simulink model "hdlcoder_fft40"  (R2026a)
settings: Solver=FixedStepDiscrete  StopTime=stoptime
PostLoadFcn:
  | load('fft40_vars.mat')
values from neighbouring files (symbols this model uses):
  N = 40    [fft40_vars.mat]
undefined symbols (not defined in the file or in its folder): TWIDDLE
libraries: dsphdlxfrm x5, dspsrcs4 x2
settings Model: DataTypeOverride=Off  Creator=The MathWorks, Inc.  LastModifiedBy=The MathWorks, Inc.
settings OptimizationCC: ConditionallyExecuteInputs=off
settings DebuggingCC: SignalRangeChecking=warning  AlgebraicLoopMsg=error  SingleTaskRateTransMsg=error  PregeneratedLibrarySubsystemCodeDiagnostic=none
settings HardwareCC: ProdHWDeviceType=ASIC/FPGA->ASIC/FPGA  TargetBitPerLong=64.0  TargetBitPerPointer=64.0  TargetBitPerSizeT=64.0  TargetBitPerPtrDiffT=64.0  TargetLongLongMode=on  TargetIntDivRoundTo=Zero  TargetEndianess=LittleEndian  TargetWordSize=64.0  TargetHWDeviceType=Custom Processor->MATLAB Host Computer  ProdEqTarget=off

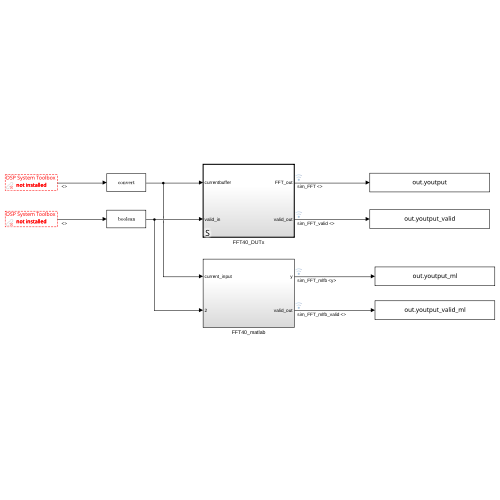
[thumbnail: Simulink's stored preview of the top-level diagram]
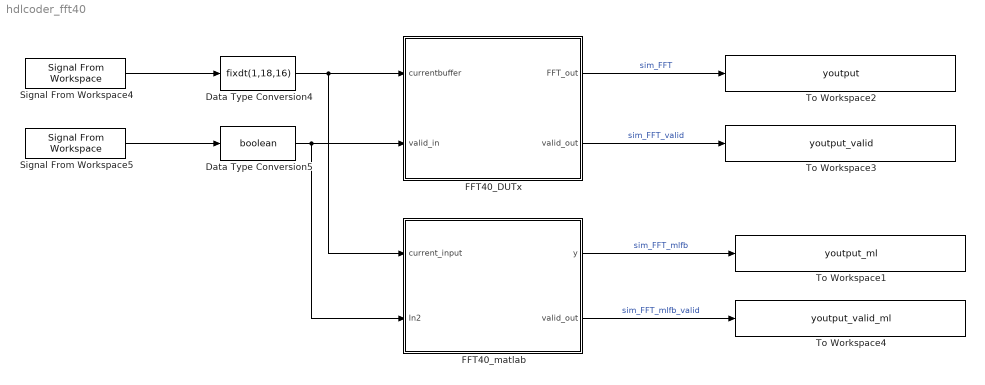
== system hdlcoder_fft40 ==
  Data Type Conversion4 : DataTypeConversion  OutDataTypeStr=fixdt(1,18,16)  SaturateOnIntegerOverflow=off  RndMeth=Floor
  Data Type Conversion5 : DataTypeConversion  OutDataTypeStr=boolean  SaturateOnIntegerOverflow=off  RndMeth=Floor
  FFT40_DUTx : Subsystem
  FFT40_matlab : Subsystem
  Signal From Workspace4 : dspsrcs4/Signal From Workspace  X=xinput  Ts=1/N  nsamps=N  OutputAfterFinalValue=Setting to zero  ignoreOrWarnInputAndFrameLengths=off  OutputFrames=off
  Signal From Workspace5 : dspsrcs4/Signal From Workspace  X=xvalid  Ts=1  nsamps=1  OutputAfterFinalValue=Holding final value  ignoreOrWarnInputAndFrameLengths=off  OutputFrames=off
  To Workspace1 : ToWorkspace  VariableName=youtput_ml  SampleTime=-1
  To Workspace2 : ToWorkspace  VariableName=youtput  SampleTime=-1
  To Workspace3 : ToWorkspace  VariableName=youtput_valid  SampleTime=-1
  To Workspace4 : ToWorkspace  VariableName=youtput_valid_ml  SampleTime=-1
  wires:
  Data Type Conversion5/1 -> FFT40_matlab/2(In2), FFT40_DUTx/2(valid_in)
  Signal From Workspace5/1 -> Data Type Conversion5/1
  Data Type Conversion4/1 -> FFT40_matlab/1(current_input), FFT40_DUTx/1(currentbuffer)
  Signal From Workspace4/1 -> Data Type Conversion4/1
  FFT40_DUTx/2(valid_out) -> To Workspace3/1  "sim_FFT_valid"
  FFT40_DUTx/1(FFT_out) -> To Workspace2/1  "sim_FFT"
  FFT40_matlab/1(y) -> To Workspace1/1  "sim_FFT_mlfb"
  FFT40_matlab/2(valid_out) -> To Workspace4/1  "sim_FFT_mlfb_valid"

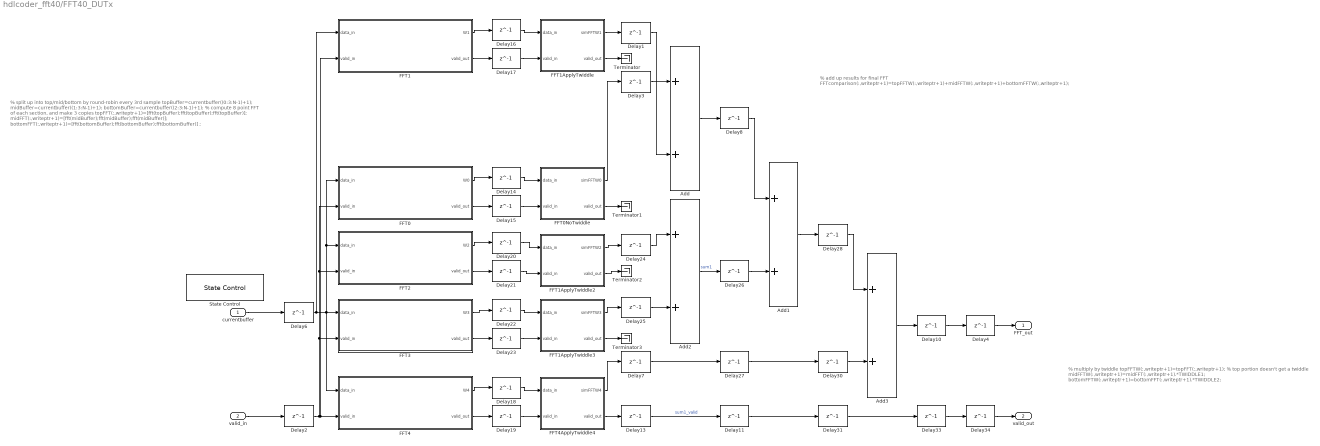
== system hdlcoder_fft40/FFT40_DUTx ==
  note: % split up into top/mid/bottom by round-robin every 3rd sample
      | topBuffer=currentbuffer((0:3:N-1)+1);
      | midBuffer=currentbuffer((1:3:N-1)+1);
      | bottomBuffer=currentbuffer((2:3:N-1)+1);
      |
      | % compute 8 point FFT of each section, and make 3 copies
      | topFFT(:,writeptr+1)=[fft(topBuffer);fft(topBuffer);fft(topBuffer)];
      | midFFT(:,writeptr+1)=[fft(midBuffer);fft(midBuffer);fft(midBuffer)];
      | bottomFFT(:,writeptr+1)=[fft(bottomBuffer);fft(bottomBuffer);fft(bottomBuffer)] ;
  note: % multiply by twiddle
      | topFFTW(:,writeptr+1)=topFFT(:,writeptr+1); % top portion doesn't get a twiddle
      | midFFTW(:,writeptr+1)=midFFT(:,writeptr+1).*TWIDDLE1;
      | bottomFFTW(:,writeptr+1)=bottomFFT(:,writeptr+1).*TWIDDLE2;
  note: % add up results for final FFT
      | FFTcomparison(:,writeptr+1)=topFFTW(:,writeptr+1)+midFFTW(:,writeptr+1)+bottomFFTW(:,writeptr+1);
  currentbuffer : Inport
  valid_in : Inport  Port=2
  Add{,1..3} (4 alike) : Sum
  Delay{1..4,6..8,10..11,13..28,30..31,33..34} (29 alike) : Delay  DelayLength=1  InitialCondition=0  UseCircularBuffer=on
  FFT0 : Subsystem
  FFT0NoTwiddle : Subsystem
  FFT1 : Subsystem
  FFT1ApplyTwiddle : Subsystem
  FFT1ApplyTwiddle2 : Subsystem
  FFT1ApplyTwiddle3 : Subsystem
  FFT2 : Subsystem
  FFT3 : Subsystem
  FFT4 : Subsystem
  FFT4ApplyTwiddle4 : Subsystem
  State Control : StateControl  StateControl=Synchronous
  Terminator{,1..3} (4 alike) : Terminator
  FFT_out : Outport
  valid_out : Outport  Port=2
  wires:
  Delay19/1 -> FFT4ApplyTwiddle4/2(valid_in)
  FFT4/1(W4) -> Delay18/1
  Delay20/1 -> FFT1ApplyTwiddle2/1(data_in)
  Add2/1 -> Delay26/1  "sum1"
  Delay1/1 -> Add/2
  Delay25/1 -> Add2/2
  Delay26/1 -> Add1/2
  Delay33/1 -> Delay34/1
  Add3/1 -> Delay10/1
  Delay24/1 -> Add2/1
  FFT3/2(valid_out) -> Delay23/1
  Delay2/1 -> FFT1/2(valid_in), FFT4/2(valid_in), FFT2/2(valid_in), FFT0/2(valid_in), FFT3/2(valid_in)
  FFT2/1(W2) -> Delay20/1
  Delay23/1 -> FFT1ApplyTwiddle3/2(valid_in)
  FFT1/2(valid_out) -> Delay17/1
  currentbuffer/1 -> Delay6/1
  FFT1ApplyTwiddle3/2(valid_out) -> Terminator3/1
  FFT1ApplyTwiddle2/2(valid_out) -> Terminator2/1
  Delay15/1 -> FFT0NoTwiddle/2(valid_in)
  FFT0NoTwiddle/2(valid_out) -> Terminator1/1
  FFT3/1(W3) -> Delay22/1
  FFT1ApplyTwiddle3/1(simFFTW3) -> Delay25/1
  FFT1ApplyTwiddle/2(valid_out) -> Terminator/1
  Delay4/1 -> FFT_out/1
  FFT1ApplyTwiddle2/1(simFFTW2) -> Delay24/1
  Delay16/1 -> FFT1ApplyTwiddle/1(data_in)
  FFT4ApplyTwiddle4/2(valid_out) -> Delay13/1
  FFT4/2(valid_out) -> Delay19/1
  Delay18/1 -> FFT4ApplyTwiddle4/1(data_in)
  Delay14/1 -> FFT0NoTwiddle/1(data_in)
  Delay10/1 -> Delay4/1
  FFT0/2(valid_out) -> Delay15/1
  valid_in/1 -> Delay2/1
  Delay8/1 -> Add1/1
  FFT4ApplyTwiddle4/1(simFFTW4) -> Delay7/1
  Delay3/1 -> Add/1
  FFT1/1(W1) -> Delay16/1
  Delay6/1 -> FFT0/1(data_in), FFT2/1(data_in), FFT3/1(data_in), FFT4/1(data_in), FFT1/1(data_in)
  FFT1ApplyTwiddle/1(simFFTW1) -> Delay1/1
  Delay17/1 -> FFT1ApplyTwiddle/2(valid_in)
  Delay21/1 -> FFT1ApplyTwiddle2/2(valid_in)
  Delay30/1 -> Add3/2
  Add1/1 -> Delay28/1
  FFT0/1(W0) -> Delay14/1
  Delay34/1 -> valid_out/1
  FFT2/2(valid_out) -> Delay21/1
  Add/1 -> Delay8/1
  Delay28/1 -> Add3/1
  Delay22/1 -> FFT1ApplyTwiddle3/1(data_in)
  FFT0NoTwiddle/1(simFFTW0) -> Delay3/1
  Delay7/1 -> Delay27/1
  Delay13/1 -> Delay11/1  "sum1_valid"
  Delay27/1 -> Delay30/1
  Delay11/1 -> Delay31/1
  Delay31/1 -> Delay33/1

== system hdlcoder_fft40/FFT40_matlab ==
  current_input : Inport
  In2 : Inport  Port=2
  fft_40 : MATLAB Function  TreatAsAtomicUnit=on
  y : Outport
  valid_out : Outport  Port=2
  wires:
  current_input/1 -> fft_40/1(x)
  In2/1 -> valid_out/1
  fft_40/1(y) -> y/1

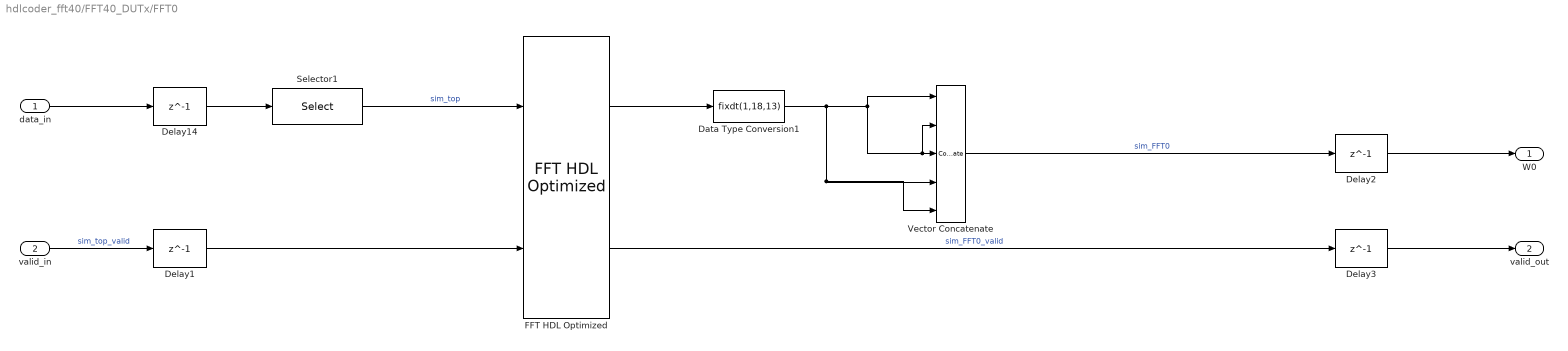
== system hdlcoder_fft40/FFT40_DUTx/FFT0 ==
  data_in : Inport
  valid_in : Inport  Port=2
  Data Type Conversion1 : DataTypeConversion  OutDataTypeStr=fixdt(1,18,13)  ConvertRealWorld=Stored Integer (SI)  SaturateOnIntegerOverflow=off  RndMeth=Floor
  Delay{1..3,14} (4 alike) : Delay  DelayLength=1  InitialCondition=0  UseCircularBuffer=on
  FFT HDL Optimized : dsphdlxfrm/FFT HDL Optimized  FFTLength=8  Architecture=Streaming Radix 2^2  ComplexMultiplication=Use 4 multipliers and 2 adders  BitReversedOutput=off  BitReversedInput=off  Normalize=on  SimulateUsing=Code generation  RoundingMethod=Floor  ResetInputPort=off  StartOutputPort=off  EndOutputPort=off
  Selector1 : Selector  IndexMode=Zero-based  InputPortWidth=N  IndexOptions=Index vector (dialog)  Indices=0:5:N-1  OutputSizes=1
  Vector Concatenate : Concatenate  NumInputs=5
  W0 : Outport
  valid_out : Outport  Port=2
  wires:
  data_in/1 -> Delay14/1
  FFT HDL Optimized/1 -> Data Type Conversion1/1
  valid_in/1 -> Delay1/1  "sim_top_valid"
  Selector1/1 -> FFT HDL Optimized/1  "sim_top"
  Vector Concatenate/1 -> Delay2/1  "sim_FFT0"
  FFT HDL Optimized/2 -> Delay3/1  "sim_FFT0_valid"
  Delay14/1 -> Selector1/1
  Delay1/1 -> FFT HDL Optimized/2
  Delay2/1 -> W0/1
  Delay3/1 -> valid_out/1
  Data Type Conversion1/1 -> Vector Concatenate/5, Vector Concatenate/4, Vector Concatenate/3, Vector Concatenate/2, Vector Concatenate/1

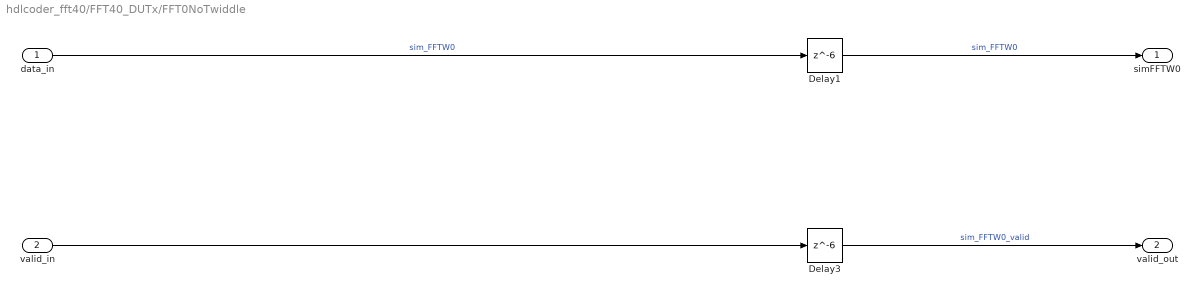
== system hdlcoder_fft40/FFT40_DUTx/FFT0NoTwiddle ==
  data_in : Inport
  valid_in : Inport  Port=2
  Delay1 : Delay  DelayLength=6
  Delay3 : Delay  DelayLength=6
  simFFTW0 : Outport
  valid_out : Outport  Port=2
  wires:
  valid_in/1 -> Delay3/1
  Delay3/1 -> valid_out/1  "sim_FFTW0_valid"
  data_in/1 -> Delay1/1  "sim_FFTW0"
  Delay1/1 -> simFFTW0/1  "sim_FFTW0"

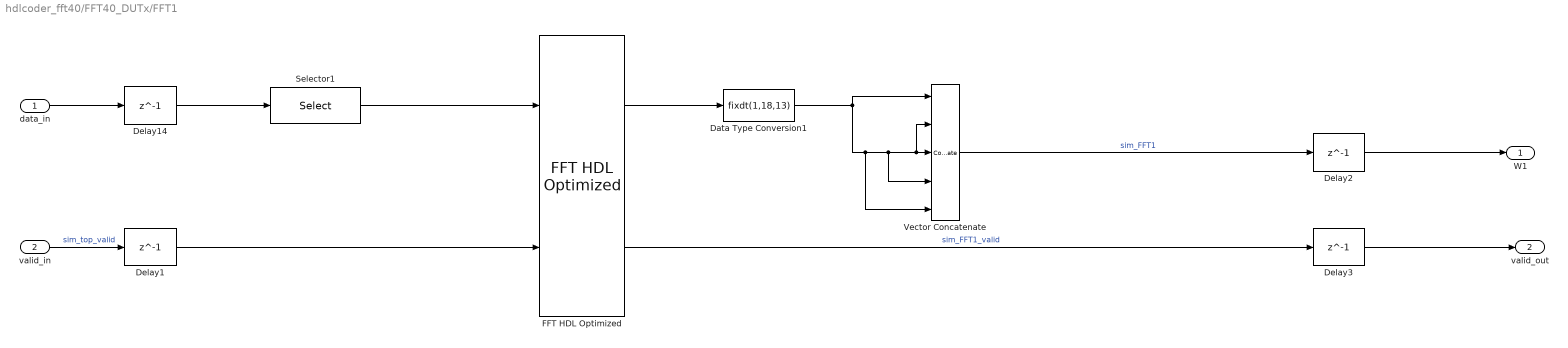
== system hdlcoder_fft40/FFT40_DUTx/FFT1 ==
  data_in : Inport
  valid_in : Inport  Port=2
  Data Type Conversion1 : DataTypeConversion  OutDataTypeStr=fixdt(1,18,13)  ConvertRealWorld=Stored Integer (SI)  SaturateOnIntegerOverflow=off  RndMeth=Floor
  Delay{1..3,14} (4 alike) : Delay  DelayLength=1  InitialCondition=0  UseCircularBuffer=on
  FFT HDL Optimized : dsphdlxfrm/FFT HDL Optimized  FFTLength=8  Architecture=Streaming Radix 2^2  ComplexMultiplication=Use 4 multipliers and 2 adders  BitReversedOutput=off  BitReversedInput=off  Normalize=on  SimulateUsing=Code generation  RoundingMethod=Floor  ResetInputPort=off  StartOutputPort=off  EndOutputPort=off
  Selector1 : Selector  IndexMode=Zero-based  InputPortWidth=N  IndexOptions=Index vector (dialog)  Indices=1:5:N-1  OutputSizes=1
  Vector Concatenate : Concatenate  NumInputs=5
  W1 : Outport
  valid_out : Outport  Port=2
  wires:
  FFT HDL Optimized/2 -> Delay3/1  "sim_FFT1_valid"
  Vector Concatenate/1 -> Delay2/1  "sim_FFT1"
  Selector1/1 -> FFT HDL Optimized/1
  valid_in/1 -> Delay1/1  "sim_top_valid"
  FFT HDL Optimized/1 -> Data Type Conversion1/1
  data_in/1 -> Delay14/1
  Delay14/1 -> Selector1/1
  Delay1/1 -> FFT HDL Optimized/2
  Delay2/1 -> W1/1
  Delay3/1 -> valid_out/1
  Data Type Conversion1/1 -> Vector Concatenate/1, Vector Concatenate/5, Vector Concatenate/4, Vector Concatenate/2, Vector Concatenate/3

== system hdlcoder_fft40/FFT40_DUTx/FFT1ApplyTwiddle ==
  data_in : Inport
  valid_in : Inport  Port=2
  ComplexMultiply : Subsystem
  Delay3 : Delay  DelayLength=6
  simFFTW1 : Outport
  valid_out : Outport  Port=2
  wires:
  ComplexMultiply/1(productout) -> simFFTW1/1  "sim_FFTW1"
  Delay3/1 -> valid_out/1  "sim_FFTW1_valid"
  data_in/1 -> ComplexMultiply/1(datin1)
  valid_in/1 -> Delay3/1

== system hdlcoder_fft40/FFT40_DUTx/FFT1ApplyTwiddle2 ==
  data_in : Inport
  valid_in : Inport  Port=2
  ComplexMultiply : Subsystem
  Delay3 : Delay  DelayLength=6
  simFFTW2 : Outport
  valid_out : Outport  Port=2
  wires:
  ComplexMultiply/1(productout) -> simFFTW2/1  "sim_FFTW2"
  Delay3/1 -> valid_out/1  "sim_FFTW2_valid"
  data_in/1 -> ComplexMultiply/1(datin1)
  valid_in/1 -> Delay3/1

== system hdlcoder_fft40/FFT40_DUTx/FFT1ApplyTwiddle3 ==
  data_in : Inport
  valid_in : Inport  Port=2
  ComplexMultiply : Subsystem
  Delay3 : Delay  DelayLength=6
  simFFTW3 : Outport
  valid_out : Outport  Port=2
  wires:
  ComplexMultiply/1(productout) -> simFFTW3/1  "sim_FFTW3"
  Delay3/1 -> valid_out/1  "sim_FFTW3_valid"
  data_in/1 -> ComplexMultiply/1(datin1)
  valid_in/1 -> Delay3/1

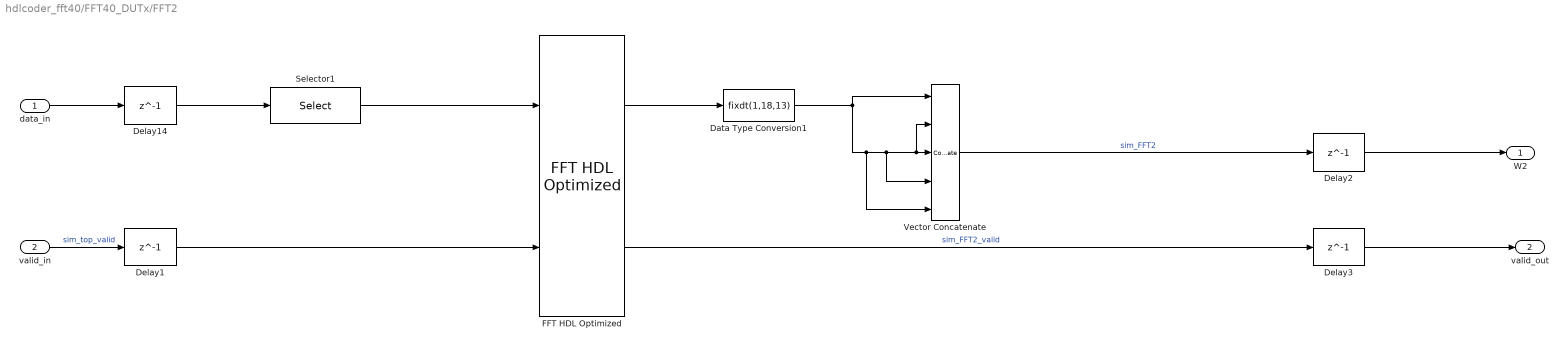
== system hdlcoder_fft40/FFT40_DUTx/FFT2 ==
  data_in : Inport
  valid_in : Inport  Port=2
  Data Type Conversion1 : DataTypeConversion  OutDataTypeStr=fixdt(1,18,13)  ConvertRealWorld=Stored Integer (SI)  SaturateOnIntegerOverflow=off  RndMeth=Floor
  Delay{1..3,14} (4 alike) : Delay  DelayLength=1  InitialCondition=0  UseCircularBuffer=on
  FFT HDL Optimized : dsphdlxfrm/FFT HDL Optimized  FFTLength=8  Architecture=Streaming Radix 2^2  ComplexMultiplication=Use 4 multipliers and 2 adders  BitReversedOutput=off  BitReversedInput=off  Normalize=on  SimulateUsing=Code generation  RoundingMethod=Floor  ResetInputPort=off  StartOutputPort=off  EndOutputPort=off
  Selector1 : Selector  IndexMode=Zero-based  InputPortWidth=N  IndexOptions=Index vector (dialog)  Indices=2:5:N-1  OutputSizes=1
  Vector Concatenate : Concatenate  NumInputs=5
  W2 : Outport
  valid_out : Outport  Port=2
  wires:
  FFT HDL Optimized/2 -> Delay3/1  "sim_FFT2_valid"
  Vector Concatenate/1 -> Delay2/1  "sim_FFT2"
  Selector1/1 -> FFT HDL Optimized/1
  valid_in/1 -> Delay1/1  "sim_top_valid"
  FFT HDL Optimized/1 -> Data Type Conversion1/1
  data_in/1 -> Delay14/1
  Delay14/1 -> Selector1/1
  Delay1/1 -> FFT HDL Optimized/2
  Delay2/1 -> W2/1
  Delay3/1 -> valid_out/1
  Data Type Conversion1/1 -> Vector Concatenate/1, Vector Concatenate/5, Vector Concatenate/4, Vector Concatenate/2, Vector Concatenate/3

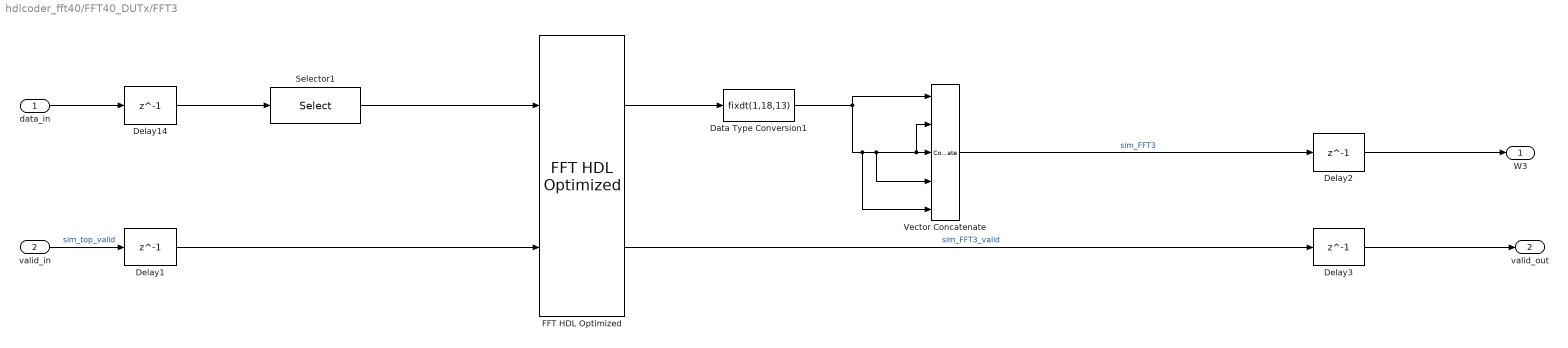
== system hdlcoder_fft40/FFT40_DUTx/FFT3 ==
  data_in : Inport
  valid_in : Inport  Port=2
  Data Type Conversion1 : DataTypeConversion  OutDataTypeStr=fixdt(1,18,13)  ConvertRealWorld=Stored Integer (SI)  SaturateOnIntegerOverflow=off  RndMeth=Floor
  Delay{1..3,14} (4 alike) : Delay  DelayLength=1  InitialCondition=0  UseCircularBuffer=on
  FFT HDL Optimized : dsphdlxfrm/FFT HDL Optimized  FFTLength=8  Architecture=Streaming Radix 2^2  ComplexMultiplication=Use 4 multipliers and 2 adders  BitReversedOutput=off  BitReversedInput=off  Normalize=on  SimulateUsing=Code generation  RoundingMethod=Floor  ResetInputPort=off  StartOutputPort=off  EndOutputPort=off
  Selector1 : Selector  IndexMode=Zero-based  InputPortWidth=N  IndexOptions=Index vector (dialog)  Indices=3:5:N-1  OutputSizes=1
  Vector Concatenate : Concatenate  NumInputs=5
  W3 : Outport
  valid_out : Outport  Port=2
  wires:
  FFT HDL Optimized/2 -> Delay3/1  "sim_FFT3_valid"
  Vector Concatenate/1 -> Delay2/1  "sim_FFT3"
  Selector1/1 -> FFT HDL Optimized/1
  valid_in/1 -> Delay1/1  "sim_top_valid"
  FFT HDL Optimized/1 -> Data Type Conversion1/1
  data_in/1 -> Delay14/1
  Delay14/1 -> Selector1/1
  Delay1/1 -> FFT HDL Optimized/2
  Delay2/1 -> W3/1
  Delay3/1 -> valid_out/1
  Data Type Conversion1/1 -> Vector Concatenate/1, Vector Concatenate/5, Vector Concatenate/4, Vector Concatenate/2, Vector Concatenate/3

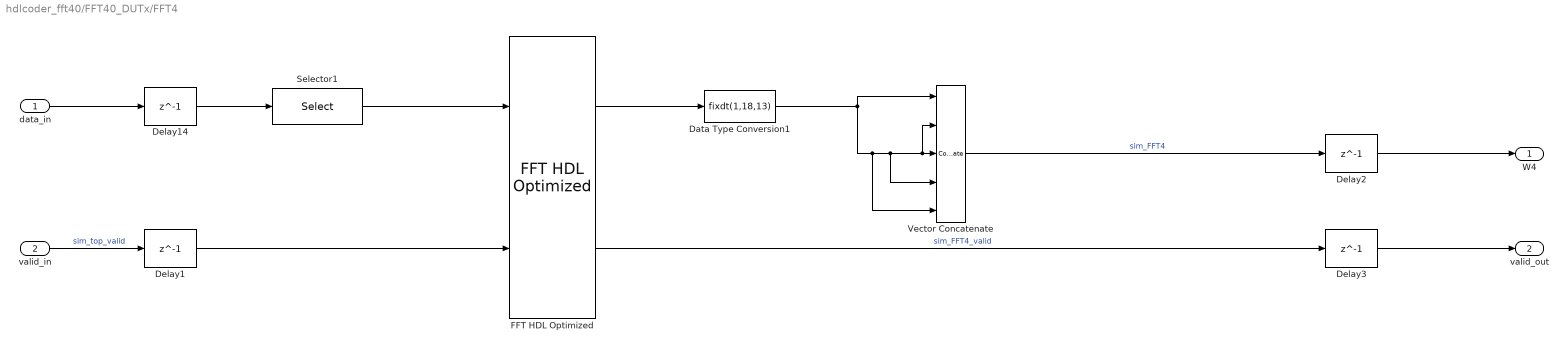
== system hdlcoder_fft40/FFT40_DUTx/FFT4 ==
  data_in : Inport
  valid_in : Inport  Port=2
  Data Type Conversion1 : DataTypeConversion  OutDataTypeStr=fixdt(1,18,13)  ConvertRealWorld=Stored Integer (SI)  SaturateOnIntegerOverflow=off  RndMeth=Floor
  Delay{1..3,14} (4 alike) : Delay  DelayLength=1  InitialCondition=0  UseCircularBuffer=on
  FFT HDL Optimized : dsphdlxfrm/FFT HDL Optimized  FFTLength=8  Architecture=Streaming Radix 2^2  ComplexMultiplication=Use 4 multipliers and 2 adders  BitReversedOutput=off  BitReversedInput=off  Normalize=on  SimulateUsing=Code generation  RoundingMethod=Floor  ResetInputPort=off  StartOutputPort=off  EndOutputPort=off
  Selector1 : Selector  IndexMode=Zero-based  InputPortWidth=N  IndexOptions=Index vector (dialog)  Indices=4:5:N-1  OutputSizes=1
  Vector Concatenate : Concatenate  NumInputs=5
  W4 : Outport
  valid_out : Outport  Port=2
  wires:
  data_in/1 -> Delay14/1
  FFT HDL Optimized/1 -> Data Type Conversion1/1
  valid_in/1 -> Delay1/1  "sim_top_valid"
  Selector1/1 -> FFT HDL Optimized/1
  Vector Concatenate/1 -> Delay2/1  "sim_FFT4"
  FFT HDL Optimized/2 -> Delay3/1  "sim_FFT4_valid"
  Delay14/1 -> Selector1/1
  Delay1/1 -> FFT HDL Optimized/2
  Delay2/1 -> W4/1
  Delay3/1 -> valid_out/1
  Data Type Conversion1/1 -> Vector Concatenate/5, Vector Concatenate/4, Vector Concatenate/3, Vector Concatenate/2, Vector Concatenate/1

== system hdlcoder_fft40/FFT40_DUTx/FFT4ApplyTwiddle4 ==
  data_in : Inport
  valid_in : Inport  Port=2
  ComplexMultiply : Subsystem
  Delay3 : Delay  DelayLength=6
  simFFTW4 : Outport
  valid_out : Outport  Port=2
  wires:
  valid_in/1 -> Delay3/1
  data_in/1 -> ComplexMultiply/1(datin1)
  Delay3/1 -> valid_out/1  "sim_FFTW4_valid"
  ComplexMultiply/1(productout) -> simFFTW4/1  "sim_FFTW4"

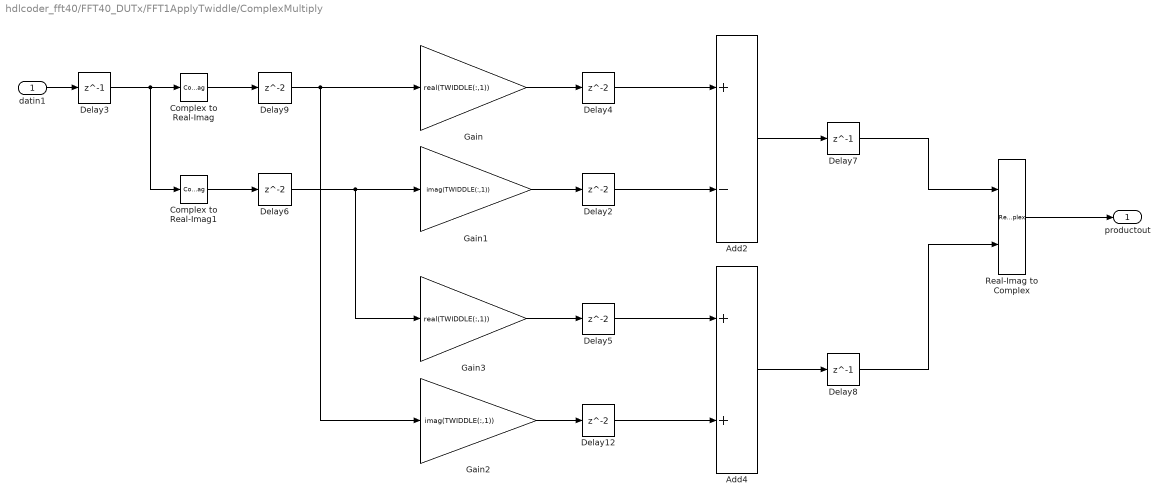
== system hdlcoder_fft40/FFT40_DUTx/FFT1ApplyTwiddle/ComplexMultiply ==
  datin1 : Inport
  Add2 : Sum  Inputs=+-
  Add4 : Sum
  Complex to Real-Imag : ComplexToRealImag  Output=Real
  Complex to Real-Imag1 : ComplexToRealImag  Output=Imag
  Delay{2,4..6,9,12} (6 alike) : Delay
  Delay3 : Delay  DelayLength=1
  Delay7 : Delay  DelayLength=1
  Delay8 : Delay  DelayLength=1
  Gain : Gain  Gain=real(TWIDDLE(:,1))  ParamDataTypeStr=fixdt(1,18,16)
  Gain1 : Gain  Gain=imag(TWIDDLE(:,1))  ParamDataTypeStr=fixdt(1,18,16)
  Gain2 : Gain  Gain=imag(TWIDDLE(:,1))  ParamDataTypeStr=fixdt(1,18,16)
  Gain3 : Gain  Gain=real(TWIDDLE(:,1))  ParamDataTypeStr=fixdt(1,18,16)
  Real-Imag to Complex : RealImagToComplex
  productout : Outport
  wires:
  datin1/1 -> Delay3/1
  Real-Imag to Complex/1 -> productout/1
  Delay3/1 -> Complex to Real-Imag/1, Complex to Real-Imag1/1
  Add2/1 -> Delay7/1
  Add4/1 -> Delay8/1
  Delay7/1 -> Real-Imag to Complex/1
  Delay8/1 -> Real-Imag to Complex/2
  Complex to Real-Imag/1 -> Delay9/1
  Complex to Real-Imag1/1 -> Delay6/1
  Delay4/1 -> Add2/1
  Delay2/1 -> Add2/2
  Delay5/1 -> Add4/1
  Delay12/1 -> Add4/2
  Gain/1 -> Delay4/1
  Gain1/1 -> Delay2/1
  Delay9/1 -> Gain2/1, Gain/1
  Delay6/1 -> Gain3/1, Gain1/1
  Gain3/1 -> Delay5/1
  Gain2/1 -> Delay12/1

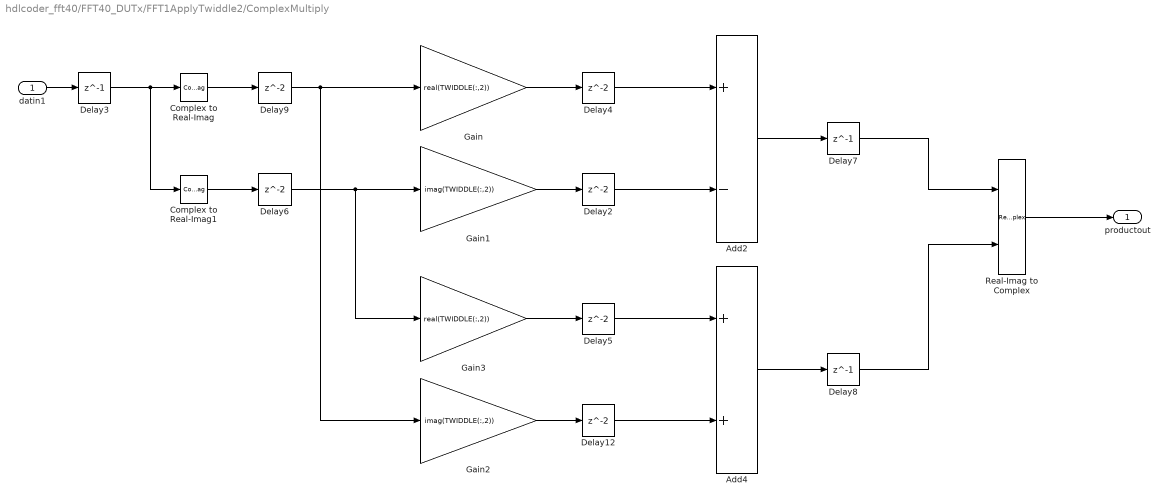
== system hdlcoder_fft40/FFT40_DUTx/FFT1ApplyTwiddle2/ComplexMultiply ==
  datin1 : Inport
  Add2 : Sum  Inputs=+-
  Add4 : Sum
  Complex to Real-Imag : ComplexToRealImag  Output=Real
  Complex to Real-Imag1 : ComplexToRealImag  Output=Imag
  Delay{2,4..6,9,12} (6 alike) : Delay
  Delay3 : Delay  DelayLength=1
  Delay7 : Delay  DelayLength=1
  Delay8 : Delay  DelayLength=1
  Gain : Gain  Gain=real(TWIDDLE(:,2))  ParamDataTypeStr=fixdt(1,18,16)
  Gain1 : Gain  Gain=imag(TWIDDLE(:,2))  ParamDataTypeStr=fixdt(1,18,16)
  Gain2 : Gain  Gain=imag(TWIDDLE(:,2))  ParamDataTypeStr=fixdt(1,18,16)
  Gain3 : Gain  Gain=real(TWIDDLE(:,2))  ParamDataTypeStr=fixdt(1,18,16)
  Real-Imag to Complex : RealImagToComplex
  productout : Outport
  wires:
  datin1/1 -> Delay3/1
  Real-Imag to Complex/1 -> productout/1
  Delay3/1 -> Complex to Real-Imag/1, Complex to Real-Imag1/1
  Add2/1 -> Delay7/1
  Add4/1 -> Delay8/1
  Delay7/1 -> Real-Imag to Complex/1
  Delay8/1 -> Real-Imag to Complex/2
  Complex to Real-Imag/1 -> Delay9/1
  Complex to Real-Imag1/1 -> Delay6/1
  Delay4/1 -> Add2/1
  Delay2/1 -> Add2/2
  Delay5/1 -> Add4/1
  Delay12/1 -> Add4/2
  Gain/1 -> Delay4/1
  Gain1/1 -> Delay2/1
  Delay9/1 -> Gain2/1, Gain/1
  Delay6/1 -> Gain3/1, Gain1/1
  Gain3/1 -> Delay5/1
  Gain2/1 -> Delay12/1

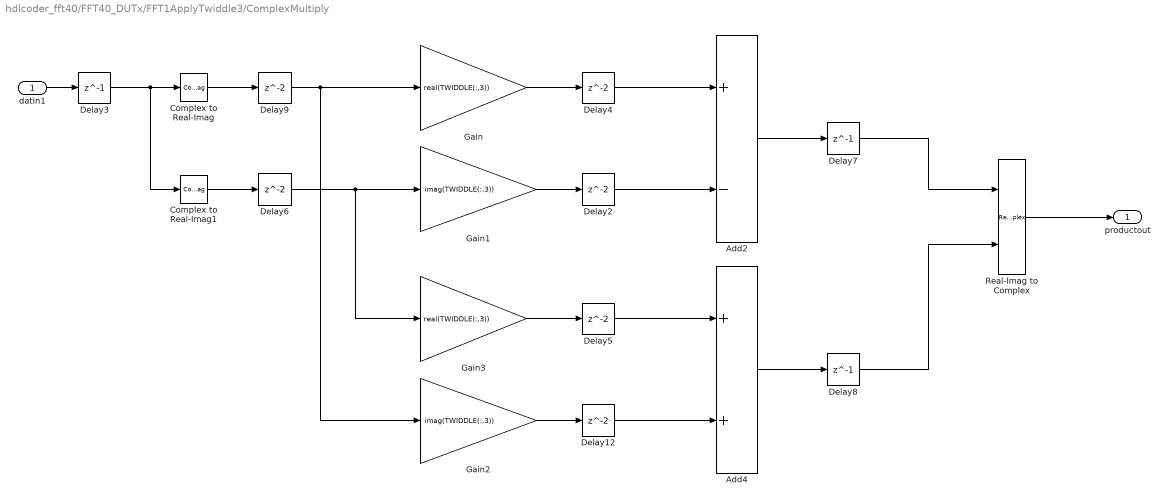
== system hdlcoder_fft40/FFT40_DUTx/FFT1ApplyTwiddle3/ComplexMultiply ==
  datin1 : Inport
  Add2 : Sum  Inputs=+-
  Add4 : Sum
  Complex to Real-Imag : ComplexToRealImag  Output=Real
  Complex to Real-Imag1 : ComplexToRealImag  Output=Imag
  Delay{2,4..6,9,12} (6 alike) : Delay
  Delay3 : Delay  DelayLength=1
  Delay7 : Delay  DelayLength=1
  Delay8 : Delay  DelayLength=1
  Gain : Gain  Gain=real(TWIDDLE(:,3))  ParamDataTypeStr=fixdt(1,18,16)
  Gain1 : Gain  Gain=imag(TWIDDLE(:,3))  ParamDataTypeStr=fixdt(1,18,16)
  Gain2 : Gain  Gain=imag(TWIDDLE(:,3))  ParamDataTypeStr=fixdt(1,18,16)
  Gain3 : Gain  Gain=real(TWIDDLE(:,3))  ParamDataTypeStr=fixdt(1,18,16)
  Real-Imag to Complex : RealImagToComplex
  productout : Outport
  wires:
  datin1/1 -> Delay3/1
  Real-Imag to Complex/1 -> productout/1
  Delay3/1 -> Complex to Real-Imag/1, Complex to Real-Imag1/1
  Add2/1 -> Delay7/1
  Add4/1 -> Delay8/1
  Delay7/1 -> Real-Imag to Complex/1
  Delay8/1 -> Real-Imag to Complex/2
  Complex to Real-Imag/1 -> Delay9/1
  Complex to Real-Imag1/1 -> Delay6/1
  Delay4/1 -> Add2/1
  Delay2/1 -> Add2/2
  Delay5/1 -> Add4/1
  Delay12/1 -> Add4/2
  Gain/1 -> Delay4/1
  Gain1/1 -> Delay2/1
  Delay9/1 -> Gain2/1, Gain/1
  Delay6/1 -> Gain3/1, Gain1/1
  Gain3/1 -> Delay5/1
  Gain2/1 -> Delay12/1

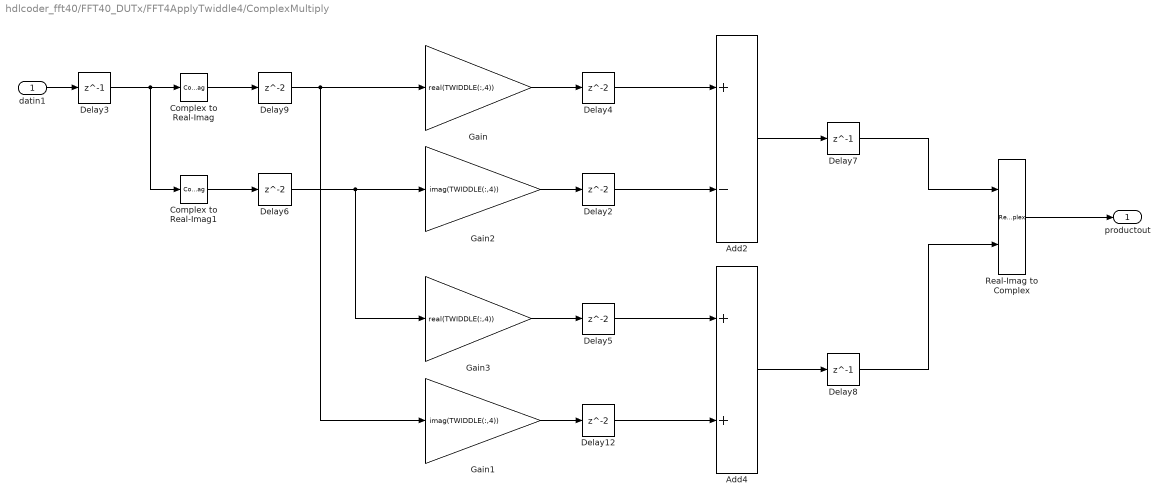
== system hdlcoder_fft40/FFT40_DUTx/FFT4ApplyTwiddle4/ComplexMultiply ==
  datin1 : Inport
  Add2 : Sum  Inputs=+-
  Add4 : Sum
  Complex to Real-Imag : ComplexToRealImag  Output=Real
  Complex to Real-Imag1 : ComplexToRealImag  Output=Imag
  Delay{2,4..6,9,12} (6 alike) : Delay
  Delay3 : Delay  DelayLength=1
  Delay7 : Delay  DelayLength=1
  Delay8 : Delay  DelayLength=1
  Gain : Gain  Gain=real(TWIDDLE(:,4))  ParamDataTypeStr=fixdt(1,18,16)
  Gain1 : Gain  Gain=imag(TWIDDLE(:,4))  ParamDataTypeStr=fixdt(1,18,16)
  Gain2 : Gain  Gain=imag(TWIDDLE(:,4))  ParamDataTypeStr=fixdt(1,18,16)
  Gain3 : Gain  Gain=real(TWIDDLE(:,4))  ParamDataTypeStr=fixdt(1,18,16)
  Real-Imag to Complex : RealImagToComplex
  productout : Outport
  wires:
  Gain1/1 -> Delay12/1
  Gain3/1 -> Delay5/1
  Delay6/1 -> Gain3/1, Gain2/1
  Delay9/1 -> Gain1/1, Gain/1
  Gain2/1 -> Delay2/1
  Gain/1 -> Delay4/1
  Delay12/1 -> Add4/2
  Delay5/1 -> Add4/1
  Delay2/1 -> Add2/2
  Delay4/1 -> Add2/1
  Complex to Real-Imag1/1 -> Delay6/1
  Complex to Real-Imag/1 -> Delay9/1
  Delay8/1 -> Real-Imag to Complex/2
  Delay7/1 -> Real-Imag to Complex/1
  Add4/1 -> Delay8/1
  Add2/1 -> Delay7/1
  Delay3/1 -> Complex to Real-Imag1/1, Complex to Real-Imag/1
  Real-Imag to Complex/1 -> productout/1
  datin1/1 -> Delay3/1

== matlab function hdlcoder_fft40/FFT40_matlab/fft_40 ==
  settings: fimath=hdlfimath
  data: x input; y output size=[40 1]; TWIDDLE parameter; N parameter
function y = fft_40(x, TWIDDLE, N)
    % split up into top/mid/bottom by round-robin every 5th sample
    Buffer0=x((0:5:N-1)+1); 
    Buffer1=x((1:5:N-1)+1); 
    Buffer2=x((2:5:N-1)+1);
    Buffer3=x((3:5:N-1)+1);
    Buffer4=x((4:5:N-1)+1);

    % compute 8 point FFT of each section
    fft0 = fft8(Buffer0);
    fft1 = fft8(Buffer1);
    fft2 = fft8(Buffer2);
    fft3 = fft8(Buffer3);
    fft4 = fft8(Buffer4);

    % make 5-copies of each 8-point fft
    FFT = [[fft0; fft0; fft0; fft0; fft0], ...
           [fft1; fft1; fft1; fft1; fft1], ...
           [fft2; fft2; fft2; fft2; fft2], ...
           [fft3; fft3; fft3; fft3; fft3], ...
           [fft4; fft4; fft4; fft4; fft4]];

    % multiply by twiddle
    FFTW0 = FFT(:,1); % top portion doesn't get a twiddle
    FFTW14 = complexGain(FFT(:,2:end), TWIDDLE);
    
    % add up results for final FFT
    t1 = coder.hdl.pipeline(FFTW0 + FFTW14(:,1));
    t2 = coder.hdl.pipeline(FFTW14(:,2) + FFTW14(:,3));
    t3 = coder.hdl.pipeline(t1 + t2);
    y = t3 + FFTW14(:,4);
end

function y  = fft8(u_r)
% 8 point FFT
% Real input and Complex output
% Cooley-Tukey
% Radix-2
% Decimation in Time

% N point FFT involves N/2 stages.
% 

N = 8;

%reverse input order
bitrevIdx = bitrevorder(1:N);
u = u_r(bitrevIdx);

y = fft_8(N, u);
end

function x = fft_8(N, u)

nt = numerictype(u);

tu1 = fft4(N, u(1:4));
tu2 = fft4(N, u(5:8));

i = 1:4;
tw = twf(N, i-1);
twu = hdlfi_mul(tu2 , tw);
x = bfly2(tu1, twu, nt);
% shift left 3 bits to scale by 8
x = reinterpretcast(x, numerictype(nt.SignednessBool, nt.WordLength, nt.FractionLength - 3));
end

%fft4
function x = fft4(N, u)

nt = numerictype(u);

tu1 = bfly2(u(1), u(2), nt);
tu2 = bfly2(u(3), u(4), nt);

% typical butterfly structure in an FFT
%
%    u0 --------------> tu0
%               \   /
%                \ /
%                 x
%                / \
%               /   \
%   u1 ---------------> tu1
%        tw         

i = 1:2;
tw = twf(N, (i-1)*2);
twu = hdlfi_mul(tu2 , tw);
x = bfly2(tu1, twu, nt);
end


function x = bfly2(u, v, nt)
% Two element butterfly
% use sum_fm and sum_nt to clamp the result of addition

tAdd = coder.hdl.pipeline(u + v);
tSub = coder.hdl.pipeline(u - v);
x = fi([bitshift(tAdd, -1); bitshift(tSub, -1)], nt, hdlfimath);
end

function out = hdlfi_mul(in1, in2)
% Complex fi multiplication
% use mul_fm and mul_nt to clamp the result of multiplication
re_u = real(in1);
im_u = imag(in1);

re_v = real(in2);
im_v = imag(in2);

re_re = coder.nullcopy(zeros(size(in1), 'like', re_u));
im_im = coder.nullcopy(zeros(size(in1), 'like', re_u));
re_im = coder.nullcopy(zeros(size(in1), 'like', re_u));
im_re = coder.nullcopy(zeros(size(in1), 'like', re_u));
coder.unroll();
for ii = 1:numel(in1)
    if re_v(ii) == 0
        re_re(ii) = 0;
        im_re(ii) = 0;
    elseif re_v(ii) == 1
        re_re(ii) = re_u(ii);
        im_re(ii) = im_u(ii);
    elseif re_v(ii) == -1
        re_re(ii) = uminus(re_u(ii));
        im_re(ii) = uminus(im_u(ii));
    else
        re_re(ii) = re_u(ii) * re_v(ii);
        im_re(ii) = im_u(ii) * re_v(ii);
    end
    
    if im_v(ii) == 0
        im_im(ii) = 0;
        re_im(ii) = 0;
    elseif im_v(ii) == 1
        im_im(ii) = im_u(ii);
        re_im(ii) = re_u(ii);
    elseif im_v(ii) == -1
        im_im(ii) = uminus(im_u(ii));
        re_im(ii) = uminus(re_u(ii));
    else
        im_im(ii) = im_u(ii) * im_v(ii);
        re_im(ii) = re_u(ii) * im_v(ii);
    end
end
re_re = coder.hdl.pipeline(re_re);
im_im = coder.hdl.pipeline(im_im);
re_im = coder.hdl.pipeline(re_im);
im_re = coder.hdl.pipeline(im_re);

y_re = coder.hdl.pipeline(fi(re_re - im_im, numerictype(in1), fimath(in1)));
y_im = coder.hdl.pipeline(fi(re_im + im_re, numerictype(in1), fimath(in1)));

out = complex(y_re, y_im);
end

function W = twf(N, k)
% complex roots of unity (N=32)
%W = exp(-2*pi*1i*k/N)

w_N = fi(exp(-2*pi*1i*(0:(N-1))/N).', hdlfimath);
W = w_N(k+1);
end

function y = complexGain(u, v)
% Full precision complex fi multiplication
coder.inline('always');

u_flat = reshape(u, 1, numel(u));
v_flat = reshape(v, 1, numel(v));

re_u = real(u_flat);
im_u = imag(u_flat);

re_v = real(v_flat);
im_v = imag(v_flat);

y_re1 = coder.hdl.pipeline(re_u .* re_v);
y_re2 = coder.hdl.pipeline(im_u .* im_v);

y_im1 = coder.hdl.pipeline(re_u .* im_v);
y_im2 = coder.hdl.pipeline(im_u .* re_v);

y_re = coder.hdl.pipeline(y_re1 - y_re2);
y_im = coder.hdl.pipeline(y_im1 + y_im2);

y = reshape(complex(y_re, y_im), size(u));
end
